simulink model "WaveStar"  (R2018b)
settings: Solver=ode4  StartTime=0  StopTime=141.2  FixedStep=0.001  MaxStep=0.001  RelTol=1e-3  EnableMultiTasking=on
values from neighbouring files (symbols this model uses):
  cc = 10.0    (= 10)    [controller_init.m]
  kc = 0    [controller_init.m]
  L_AB = 0.412    [controller_init.m]
  L_AC = 0.2    [controller_init.m]
  mc = 0    [controller_init.m]
  McSat = inf    [controller_init.m]
  simu = simulationClass()    [wecSimInputFile.m]
  waves = waveClass('irregular')    [wecSimInputFile.m]
  xPcTs = 0.001    [controller_init.m]
undefined symbols (not defined in the file or in its folder): body, constraint, HPfreq, LPfreq, pto, X, Y, Z
libraries: nesl_utility x72, sm_lib x38, WECSim_Lib x7, simulink x2, vrlib x1
(part 4 of 4)

== matlab function WaveStar/Controller/Rotary/lin2rot conversion/Linear2Angular Conversion/MATLAB Function1 K [m] ==
  data: u input; y output; L_AB parameter; L_AC parameter
function y = fcn(u,L_AB,L_AC)
%#codegen
y = L_AB'*L_AC'*sin(u);

== matlab function WaveStar/Controller/Linear/WECCCOMP Controller/lin2rot conversion/Linear2Angular Conversion/MATLAB Function1 a_CAB [rad] ==
  data: u input; y output; L_AB parameter; L_AC parameter
function y = fcn(u,L_AB,L_AC)
%#codegen
%
y = acos((u.^2-L_AB'^2-L_AC'^2)/(-2*L_AB'*L_AC'));

== matlab function WaveStar/C_Revolute/MATLAB Function ==
  data: vel input; t output; brkwy_trq parameter double; brkwy_vel parameter double; Col_trq parameter double; visc_coef parameter double
function t = friction(vel,brkwy_trq, brkwy_vel, Col_trq, visc_coef)
    w = -vel(5);

    %{
    brkwy_trq = .25;         % Breakaway friction torque
    brkwy_vel = 0.1;        % Breakaway friction velocity
    Col_trq = .20;           % Coulomb friction torque
    visc_coef = 0.001;      % Viscous friction coefficient
    %}
    
    static_scale = sqrt(2*exp(1))*(brkwy_trq-Col_trq);  % Scale factor for static torque
    static_thr = sqrt(2)*brkwy_vel;                     % Velocity threshold for static torque
    Col_thr = brkwy_vel/10;                             % Velocity threshold for Coulomb torque
    
    t = visc_coef * w ...
         + static_scale * (w/static_thr*exp(-(w/static_thr)^2)) ...
         + Col_trq * tanh(w/Col_thr);
end

%{
parameters
    brkwy_trq = { 25, 'N*m' };          % Breakaway friction torque
    brkwy_vel = { 0.1, 'rad/s' };       % Breakaway friction velocity
    Col_trq = { 20, 'N*m' };            % Coulomb friction torque
    visc_coef = { 0.001, 'N*m*s/rad' }; % Viscous friction coefficient
end

parameters (Access=private)
    static_scale = sqrt(2*exp(1))*(brkwy_trq-Col_trq);  % Scale factor for static torque
    static_thr = sqrt(2)*brkwy_vel;                     % Velocity threshold for static torque
    Col_thr = brkwy_vel/10;                             % Velocity threshold for Coulomb torque
end

equations
    % Parameter range checking
    assert(brkwy_trq>0)
    assert(brkwy_vel>0)
    assert(Col_trq>0)
    assert(Col_trq<=brkwy_trq)
    assert(visc_coef>=0)
    % Torque is a combination of viscous, static, and Coulomb losses
    t == visc_coef * w ...
         + static_scale * (w/static_thr*exp(-(w/static_thr)^2)) ...
         + Col_trq * tanh(w/Col_thr);
end
%}

== matlab function WaveStar/B_Revolute/MATLAB Function ==
  data: vel input; t output; brkwy_trq parameter double; brkwy_vel parameter double; Col_trq parameter double; visc_coef parameter double
function t = friction(vel,brkwy_trq, brkwy_vel, Col_trq, visc_coef)
    w = -vel(5);

    %{
    brkwy_trq = .25;         % Breakaway friction torque
    brkwy_vel = 0.1;        % Breakaway friction velocity
    Col_trq = .20;           % Coulomb friction torque
    visc_coef = 0.001;      % Viscous friction coefficient
    %}
    
    static_scale = sqrt(2*exp(1))*(brkwy_trq-Col_trq);  % Scale factor for static torque
    static_thr = sqrt(2)*brkwy_vel;                     % Velocity threshold for static torque
    Col_thr = brkwy_vel/10;                             % Velocity threshold for Coulomb torque
    
    t = visc_coef * w ...
         + static_scale * (w/static_thr*exp(-(w/static_thr)^2)) ...
         + Col_trq * tanh(w/Col_thr);
end

%{
parameters
    brkwy_trq = { 25, 'N*m' };          % Breakaway friction torque
    brkwy_vel = { 0.1, 'rad/s' };       % Breakaway friction velocity
    Col_trq = { 20, 'N*m' };            % Coulomb friction torque
    visc_coef = { 0.001, 'N*m*s/rad' }; % Viscous friction coefficient
end

parameters (Access=private)
    static_scale = sqrt(2*exp(1))*(brkwy_trq-Col_trq);  % Scale factor for static torque
    static_thr = sqrt(2)*brkwy_vel;                     % Velocity threshold for static torque
    Col_thr = brkwy_vel/10;                             % Velocity threshold for Coulomb torque
end

equations
    % Parameter range checking
    assert(brkwy_trq>0)
    assert(brkwy_vel>0)
    assert(Col_trq>0)
    assert(Col_trq<=brkwy_trq)
    assert(visc_coef>=0)
    % Torque is a combination of viscous, static, and Coulomb losses
    t == visc_coef * w ...
         + static_scale * (w/static_thr*exp(-(w/static_thr)^2)) ...
         + Col_trq * tanh(w/Col_thr);
end
%}

== matlab function WaveStar/Controller/Rotary/MATLAB Function ==
  data: ws1 input; WS1 output; ws2 input; ws3 input; float_accel input; WS2 output; WS3 output; ACC output; time input; pos input; POS output
function [WS1,WS2,WS3,ACC,POS] = addfault(ws1, ws2, ws3, float_accel, time, pos)
 
%% Wave Gauge 1
bias = 0;
drift = 0;
pDrop = 0.2; %0.3;
x = rand;
rn = 0.002*randn; %0.002*randn;
if x<pDrop
    WS1 = 0;
else
    WS1 = ws1+bias+drift*time+rn;
end
 
%% Wave Gauge 2
bias = 0;
drift = 0;
pDrop = 0.18; %0.15;
x = rand;
rn = 0.002*randn; %0.002*randn;
if x<pDrop
    WS2 = 0;
else
    WS2 = ws2+bias+drift*time+rn;
end

 
%% Wave Gauge 3
bias = 0;
drift = 0;
pDrop = 0.15; %0.2;
x = rand;
rn = 0.002*randn; %0.002*randn;
if x<pDrop
    WS3 = 0;
else
    WS3 = ws3+bias+drift*time+rn;
end
 
%% Accelerometer
bias = 0;
drift = 0;
pDrop = 0.08; %0.23;
x = rand;
rn = 0.25*randn; %0.25*randn;
if x<pDrop
    ACC = 0;
else
    ACC = float_accel+bias+drift*time+rn;
end

%% Position
bias = 0;
drift = 0;
pDrop = 0.03; %0.01;
x = rand;
rn = 0.003*randn; %0.003*randn;

if x<pDrop
    POS = 0;
else
    POS = pos+bias+drift*time+rn;
end

== matlab function WaveStar/A_Revolute/MATLAB Function ==
  data: time input; vel input; t output; brkwy_trq parameter double; brkwy_vel parameter double; Col_trq parameter double; visc_coef parameter double
function t = friction(time,vel,brkwy_trq, brkwy_vel, Col_trq, visc_coef)
    w = -vel(5);

    %{
    brkwy_trq = .25;         % Breakaway friction torque
    brkwy_vel = 0.1;        % Breakaway friction velocity
    Col_trq = .20;           % Coulomb friction torque
    visc_coef = 0.001;      % Viscous friction coefficient
    %}
    
    static_scale = sqrt(2*exp(1))*(brkwy_trq-Col_trq);  % Scale factor for static torque
    static_thr = sqrt(2)*brkwy_vel;                     % Velocity threshold for static torque
    Col_thr = brkwy_vel/10;                             % Velocity threshold for Coulomb torque
    
    if (55 < time)&&(time < 115)
    t = visc_coef * w ...
         + static_scale * (w/static_thr*exp(-(w/static_thr)^2)) ...
         + Col_trq * tanh(w/Col_thr);
    else
        t = 0;
    end
end

%{
parameters
    brkwy_trq = { 25, 'N*m' };          % Breakaway friction torque
    brkwy_vel = { 0.1, 'rad/s' };       % Breakaway friction velocity
    Col_trq = { 20, 'N*m' };            % Coulomb friction torque
    visc_coef = { 0.001, 'N*m*s/rad' }; % Viscous friction coefficient
end

parameters (Access=private)
    static_scale = sqrt(2*exp(1))*(brkwy_trq-Col_trq);  % Scale factor for static torque
    static_thr = sqrt(2)*brkwy_vel;                     % Velocity threshold for static torque
    Col_thr = brkwy_vel/10;                             % Velocity threshold for Coulomb torque
end

equations
    % Parameter range checking
    assert(brkwy_trq>0)
    assert(brkwy_vel>0)
    assert(Col_trq>0)
    assert(Col_trq<=brkwy_trq)
    assert(visc_coef>=0)
    % Torque is a combination of viscous, static, and Coulomb losses
    t == visc_coef * w ...
         + static_scale * (w/static_thr*exp(-(w/static_thr)^2)) ...
         + Col_trq * tanh(w/Col_thr);
end
%}

== matlab function WaveStar/Float/Hydrodynamic Body/Hydrostatic Restoring Force Calculation/Linear and Nonlinear Restoring Force Variant Subsystem/Nonlinear Hydrostatic Restoring Force/Restoring Forces ==
  data: x input; elv input; center input; f output; tnorm input; area input; rho input; g input; cg input; p output; mass input
function [f,p]  = nonLinearBuoyancy(x,elv,center,tnorm,area,rho,g,cg,mass)
% Function to calculate buoyancy force and moment on a triangulated surface
% NOTE: This function assumes that the STL file is imported with its CG at 0,0,0
[f,p] = calc_buoyancy(x,elv,center,tnorm,area,rho,g,cg);
f = -f + [0 0 g*mass 0 0 0]';
end


function [f,p] = calc_buoyancy(x,elv,center,tnorm,area,rho,g,cg)
% Function to apply translation and rotation and calculate forces

% Compute new tri coords after cog rotation and translation
center = rotateXYZ(center,[1 0 0],x(4));
center = rotateXYZ(center,[0 1 0],x(5));
center = rotateXYZ(center,[0 0 1],x(6));
center = offsetXYZ(center,x);
center = offsetXYZ(center,cg);
% Compute new normal vectors coords after cog rotation
tnorm = rotateXYZ(tnorm,[1 0 0],x(4));
tnorm = rotateXYZ(tnorm,[0 1 0],x(5));
tnorm = rotateXYZ(tnorm,[0 0 1],x(6));

% Calculate the hydrostatic forces
av = tnorm .* [area area area];
[f,p]=fHydrostatic(center,elv,x(1:3)+cg,av,rho,g);
end

function verts = offsetXYZ(verts,x)
% Function to move the position vertices
verts(:,1) = verts(:,1) + x(1);
verts(:,2) = verts(:,2) + x(2);
verts(:,3) = verts(:,3) + x(3);
end

function xn = rotateXYZ(x,ax,t)
% Function to rotate a point about an arbitrary axis
% x: 3-componenet coordiantes
% ax: axis about which to rotate (must be a vector length 1)
% t: rotation angle
% xn: new coordinates after rotation
rotMat = zeros(3);
rotMat(1,1) = ax(1)*ax(1)*(1-cos(t))    + cos(t);
rotMat(1,2) = ax(2)*ax(1)*(1-cos(t))    + ax(3)*sin(t);
rotMat(1,3) = ax(3)*ax(1)*(1-cos(t))    - ax(2)*sin(t);
rotMat(2,1) = ax(1)*ax(2)*(1-cos(t))    - ax(3)*sin(t);
rotMat(2,2) = ax(2)*ax(2)*(1-cos(t))    + cos(t);
rotMat(2,3) = ax(3)*ax(2)*(1-cos(t))    + ax(1)*sin(t);
rotMat(3,1) = ax(1)*ax(3)*(1-cos(t))    + ax(2)*sin(t);
rotMat(3,2) = ax(2)*ax(3)*(1-cos(t))    - ax(1)*sin(t);
rotMat(3,3) = ax(3)*ax(3)*(1-cos(t))    + cos(t);
xn = x*rotMat;
end

function [f,p] = fHydrostatic(center,elv,instcg,av,rho,g)
% Function to calculate the force and moment about the cog due to hydrostatic pressure
f = zeros(6,1);

% Zeor out regions above the mean free surface
z=center(:,3); z((z-elv)>0)=0;

% Calculate the hydrostatic pressure at each triangle center
pressureVect = rho*g.*[-z -z -z].*-av;
p = rho*g.*-z;
% Compute force about cog
f(1:3) = sum(pressureVect);

tmp1 = ones(length(center(:,1)),1);
tmp2 = tmp1*instcg';
center2cgVec = center-tmp2;

f(4:6)= sum(cross(center2cgVec,pressureVect));
end

== matlab function WaveStar/Controller/Rotary/lin2rot conversion/Linear2Angular Conversion/MATLAB Function1 L_BC [m] ==
  data: u input; y output; L_BC_neutral parameter
 function y = fcn(u,L_BC_neutral)
%#codegen
%
y = u+L_BC_neutral';

== matlab function WaveStar/Controller/Rotary/lin2rot conversion/Linear2Angular Conversion/MATLAB Function1 Theta [rad] ==
  data: u input; y output; a_CAB_neutral parameter
function y = fcn(u,a_CAB_neutral)
%#codegen
y = u-a_CAB_neutral';

== matlab function WaveStar/Controller/Rotary/lin2rot conversion/Linear2Angular Conversion/MATLAB Function1 a_CAB [rad] ==
  data: u input; y output; L_AB parameter; L_AC parameter
function y = fcn(u,L_AB,L_AC)
%#codegen
%
y = acos((u.^2-L_AB'^2-L_AC'^2)/(-2*L_AB'*L_AC'));

== matlab function WaveStar/Float/Hydrodynamic Body/Morison Element and ViscousDampingForceCalculation/Morison Element Variant Subsystem/Morison Element On/Irregular Wave Morison Force/MorrisonElement(s)  ==
  data: r input; f output; Vel input; Accel input; Disp input; Area input; Cd input; Vol input; Ca input; Time input; rho input; waveDir input; waterDepth input; k input; w input; A input; rampTime input; g input; randPhase input; dw input; currentSpeed input; currentDirection input; currentDepth input; currentOption input
function f = fcn(r,Vel,Accel,Disp,Area,Cd,Vol,Ca,Time,rho,waveDir,waterDepth,k,w,A,rampTime,g,randPhase,dw,currentSpeed,currentDirection,currentDepth,currentOption)
[rr,~]  = size(r); [ff]    = length(w);
FMt     = zeros(rr,6);
uVt     = zeros(ff,1); vVt = uVt; wVt = vVt; uAt = wVt; vAt = uAt; wAt = vAt;
for ii = 1:rr
    % Calculate Rotation Matrix
    RotMax = [cos(Disp(5))*cos(Disp(6)) , cos(Disp(4))*sin(Disp(6)) + sin(Disp(4))*sin(Disp(5))*cos(Disp(6)) , sin(Disp(4))*sin(Disp(6)) - cos(Disp(4))*sin(Disp(5))*sin(Disp(6));...
              -cos(Disp(5))*sin(Disp(6)), cos(Disp(4))*cos(Disp(6)) -  sin(Disp(4))*sin(Disp(5))*sin(Disp(6)), sin(Disp(4))*cos(Disp(6)) + cos(Disp(4))*sin(Disp(5))*sin(Disp(6));...
              sin(Disp(5))              , -sin(Disp(4))*cos(Disp(5))                                         , cos(Disp(4))*cos(Disp(5))                                        ];
    % Rotate Cartesian
    rRot    = mtimes(r(ii,:),RotMax);
    Dispt   = [Disp(1),Disp(2),Disp(3)];
    ShiftCg = Dispt + rRot;
    % Update translational and rotational velocity
    % w refers to \omega = rotational velocity
    Velt    = [Vel(4),Vel(5),Vel(6)];
    wxr     = cross(Velt,r(ii,:));
    %
    switch currentOption
        case 0
            currentSpeedDepth = currentSpeed;
        case 1
            if ShiftCg(3) > -currentDepth
                currentSpeedDepth = currentSpeed*(1 + ShiftCg(3)/currentDepth)^(1/7);
            else
                currentSpeedDepth = 0;
            end
        case 2
            if ShiftCg(3) > -currentDepth
                currentSpeedDepth = currentSpeed*(1 + ShiftCg(3)/currentDepth);
            else
                currentSpeedDepth = 0;
            end
        otherwise
            currentSpeedDepth = 0;
    end
    % Ramp Time
    if Time <= rampTime
        curramp        = currentSpeedDepth*(1 + cos(pi + pi/rampTime*Time))/2;
    else
        curramp        = currentSpeedDepth;
    end
    %Vel should be a column vector
    Vel2    = [Vel(1),Vel(2),Vel(3)] + wxr + [curramp*cosd(currentDirection),curramp*sind(currentDirection),0];
    % Update translational and rotational acceleration
    % dotw refers to \dot{\omega} = rotational acceleration
    Accelt  = [Accel(4),Accel(5),Accel(6)];
    dotwxr  = cross(Accelt,r(ii,:));
    wxwxr   = cross(Velt,wxr);
    % Update Translational Acceleration
    Accel2  = [Accel(1),Accel(2),Accel(3)] + dotwxr + wxwxr;
    %% Calculate Orbital Velocity
    for jj = 1:ff
        waveDirRad      = waveDir*pi/180;
        phaseArg        = w(jj,1)*Time - k(jj,1)*(ShiftCg(1)*cos(waveDirRad) + ShiftCg(2)*sin(waveDirRad)) + randPhase(jj,1);
        % Vertical Variation
        kh              = k(jj,1)*waterDepth;
        kz              = k(jj,1)*ShiftCg(3);
        if kh > pi % Deep Water Wave
            coeffHorz  = exp(kz);
            coeffVert  = coeffHorz;
        else % Shallow & Intermediate depth
            coeffHorz  = cosh(kz + kh)/cosh(kh);
            coeffVert  = sinh(kz + kh)/cosh(kh);
        end
        % Ramp Time
        if Time <= rampTime
            ramp        = (sqrt(A(jj,1)*dw(jj,1))/2)*(1 + cos(pi + pi/rampTime*Time));
        else
            ramp        = sqrt(A(jj,1)*dw(jj,1));
        end
        % Orbital Velocity for each individual wave component
        uVt(jj,1)       =  ramp*coeffHorz*cos(phaseArg)*g*k(jj,1)*(1/w(jj,1))*cos(waveDirRad);
        vVt(jj,1)       =  ramp*coeffHorz*cos(phaseArg)*g*k(jj,1)*(1/w(jj,1))*sin(waveDirRad);
        wVt(jj,1)       = -ramp*coeffVert*sin(phaseArg)*g*k(jj,1)*(1/w(jj,1));
        % Orbital Acceleration for each individual wave component
        uAt(jj,1)       = -ramp*coeffHorz*sin(phaseArg)*g*k(jj,1)*cos(waveDirRad);
        vAt(jj,1)       = -ramp*coeffHorz*sin(phaseArg)*g*k(jj,1)*sin(waveDirRad);
        wAt(jj,1)       = -ramp*coeffVert*cos(phaseArg)*g*k(jj,1);
    end
    % Sum the wave components to obtain the x, y, z orbital velocities
    uV = sum(uVt); uA = sum(uAt); vV = sum(vVt); vA = sum(vAt); wV = sum(wVt); wA = sum(wAt);
    %% Added inertia and drag forces
    areaRot         = abs(mtimes(Area(ii,:),RotMax));
    CdRot           = mtimes(abs(Cd(ii,:)),RotMax);
    CaRot           = abs(mtimes(Ca(ii,:),RotMax));
    % Forces from velocity drag
    uVdiff          = uV - Vel2(1); FxuV = (1/2)*abs(uVdiff)*uVdiff*rho*CdRot(1)*areaRot(1);
    vVdiff          = vV - Vel2(2); FxvV = (1/2)*abs(vVdiff)*vVdiff*rho*CdRot(2)*areaRot(2);
    wVdiff          = wV - Vel2(3); FxwV = (1/2)*abs(wVdiff)*wVdiff*rho*CdRot(3)*areaRot(3);
    % Forces from body acceleration inertia
    uAdiff          = uA - Accel2(1); FxuA = uAdiff*rho*Vol(ii,:)*CaRot(1);
    vAdiff          = vA - Accel2(2); FxvA = vAdiff*rho*Vol(ii,:)*CaRot(2);
    wAdiff          = wA - Accel2(3); FxwA = wAdiff*rho*Vol(ii,:)*CaRot(3);
    % Forces from fluid acceleration inertia
    FxuAf           = uA*Vol(ii,:)*rho;
    FxvAf           = vA*Vol(ii,:)*rho;
    FxwAf           = wA*Vol(ii,:)*rho;
    % Combine the forces and moments
    if ShiftCg(3) > 0
        F           = [0, 0, 0];
        M           = [0, 0, 0];
        FMt(ii,:)   = [F,M];
    else
        F           = [FxuV + FxuA + FxuAf,...
            FxvV + FxvA + FxvAf,...
            FxwV + FxwA + FxwAf];
        M           = cross(rRot,F);
        FMt(ii,:)   = [F,M];
    end
end
f      = 0.* Vel;
f(1:6) = [sum(FMt(:,1));sum(FMt(:,2));sum(FMt(:,3));sum(FMt(:,4));sum(FMt(:,5));sum(FMt(:,6))];

== matlab function WaveStar/Float/Hydrodynamic Body/Morison Element and ViscousDampingForceCalculation/Morison Element Variant Subsystem/Morison Element On/No Wave Morison Force/MorrisonElement(s)  ==
  data: r input; f output; Vel input; Accel input; Disp input; Area input; Cd input; Vol input; Ca input; rho input; currentSpeed input; currentDirection input; Time input; rampTime input; currentDepth input; currentOption input
function f = fcn(r,Vel,Accel,Disp,Area,Cd,Vol,Ca,rho,currentSpeed,currentDirection,Time,rampTime,currentDepth,currentOption)
[rr,~]=size(r);
FMt = zeros(rr,6);
for ii = 1:rr
    % Calculate Rotation Matrix
    RotMax = [cos(Disp(5))*cos(Disp(6)) , cos(Disp(4))*sin(Disp(6)) + sin(Disp(4))*sin(Disp(5))*cos(Disp(6)) , sin(Disp(4))*sin(Disp(6)) - cos(Disp(4))*sin(Disp(5))*sin(Disp(6));...
             -cos(Disp(5))*sin(Disp(6)), cos(Disp(4))*cos(Disp(6)) -  sin(Disp(4))*sin(Disp(5))*sin(Disp(6)), sin(Disp(4))*cos(Disp(6)) + cos(Disp(4))*sin(Disp(5))*sin(Disp(6));...
              sin(Disp(5))              , -sin(Disp(4))*cos(Disp(5))                                         , cos(Disp(4))*cos(Disp(5))                                        ];
    % Rotate Cartesian
    rRot    = mtimes(r(ii,:),RotMax);
    Dispt   = [Disp(1),Disp(2),Disp(3)];
    ShiftCg = Dispt + rRot;
    % Update translational and rotational velocity
    Velt    = [Vel(4),Vel(5),Vel(6)];                       % w refers to \omega = rotational velocity
    wxr     = cross(Velt,r(ii,:));
    switch currentOption
        case 0
             currentSpeedDepth = currentSpeed;
        case 1
            if ShiftCg(3) > -currentDepth
                currentSpeedDepth = currentSpeed*(1 + ShiftCg(3)/currentDepth)^(1/7);
            else
                currentSpeedDepth = 0;
            end
        case 2
            if ShiftCg(3) > -currentDepth
                currentSpeedDepth = currentSpeed*(1 + ShiftCg(3)/currentDepth);
            else
                currentSpeedDepth = 0;
            end
        otherwise
             currentSpeedDepth = 0;
    end
    % Ramp Time
    if Time <= rampTime
            curramp        = currentSpeedDepth*(1 + cos(pi + pi/rampTime*Time))/2;
        else
            curramp        = currentSpeedDepth;
    end
    %Vel should be a column vector
    Vel2    = [Vel(1),Vel(2),Vel(3)] + wxr + [curramp*cosd(currentDirection),curramp*sind(currentDirection),0];
    % Update translational and rotational acceleration
    Accelt  = [Accel(4),Accel(5),Accel(6)];
    dotwxr  = cross(Accelt,r(ii,:));                        % dotw refers to \dot{\omega} = rotational acceleration
    wxwxr   = cross(Velt,wxr);
    Accel2  = [Accel(1),Accel(2),Accel(3)] + dotwxr + wxwxr;
    %% Added inertia and drag forces
    areaRot = abs(mtimes(Area(ii,:),RotMax));
    CdRot   = mtimes(abs(Cd(ii,:)),RotMax);
    CaRot   = abs(mtimes(Ca(ii,:),RotMax));
    % Forces from body velocity drag
    FxuV    = (1/2)*abs(-1*Vel2(1))*-1*Vel2(1)*rho*CdRot(1)*areaRot(1);
    FxvV    = (1/2)*abs(-1*Vel2(2))*-1*Vel2(2)*rho*CdRot(2)*areaRot(2);
    FxwV    = (1/2)*abs(-1*Vel2(3))*-1*Vel2(3)*rho*CdRot(3)*areaRot(3);
    % Forces from body acceleration inertia
    FxuA = rho*Vol(ii,:)*CaRot(1)*-1*Accel2(1);
    FxvA = rho*Vol(ii,:)*CaRot(2)*-1*Accel2(2);
    FxwA = rho*Vol(ii,:)*CaRot(3)*-1*Accel2(3);
    % Sum the force and moment contributions
    if ShiftCg(3) > 0
        FMt(ii,:)   = [0, 0, 0, 0, 0, 0];
    else
        F           = [FxuV + FxuA,...
            FxvV + FxvA,...
            FxwV + FxwA];
        M           = cross(rRot,F);
        FMt(ii,:)   = [F,M];
    end
end
f      = 0.*Vel;
f(1:6) = [sum(FMt(:,1));sum(FMt(:,2));sum(FMt(:,3));sum(FMt(:,4));sum(FMt(:,5));sum(FMt(:,6))];

== matlab function WaveStar/Float/Hydrodynamic Body/Morison Element and ViscousDampingForceCalculation/Morison Element Variant Subsystem/Morison Element On/Regular Wave Morison Force/MorrisonElement(s)  ==
  data: r input; f output; Vel input; Accel input; Disp input; Area input; Cd input; Vol input; Ca input; Time input; rho input; waveDir input; waterDepth input; k input; w input; A input; rampTime input; g input; currentSpeed input; currentDirection input; currentDepth input; currentOption input
function f = fcn(r,Vel,Accel,Disp,Area,Cd,Vol,Ca,Time,rho,waveDir,waterDepth,k,w,A,rampTime,g,currentSpeed,currentDirection,currentDepth,currentOption)
[rr,~]=size(r);
FMt = zeros(rr,6);
for ii = 1:rr
    % Calculate Rotation Matrix
    RotMax = [cos(Disp(5))*cos(Disp(6)) , cos(Disp(4))*sin(Disp(6)) + sin(Disp(4))*sin(Disp(5))*cos(Disp(6)) , sin(Disp(4))*sin(Disp(6)) - cos(Disp(4))*sin(Disp(5))*sin(Disp(6));...
             -cos(Disp(5))*sin(Disp(6)), cos(Disp(4))*cos(Disp(6)) -  sin(Disp(4))*sin(Disp(5))*sin(Disp(6)), sin(Disp(4))*cos(Disp(6)) + cos(Disp(4))*sin(Disp(5))*sin(Disp(6));...
              sin(Disp(5))              , -sin(Disp(4))*cos(Disp(5))                                         , cos(Disp(4))*cos(Disp(5))                                        ];
    % Rotate Cartesian
    rRot    = mtimes(r(ii,:),RotMax);
    Dispt   = [Disp(1),Disp(2),Disp(3)];
    ShiftCg = Dispt + rRot;
    % Update translational and rotational velocity
    % w refers to \omega = rotational velocity
    Velt    = [Vel(4),Vel(5),Vel(6)]; 
    wxr     = cross(Velt,r(ii,:));
    %
    switch currentOption
        case 0
             currentSpeedDepth = currentSpeed;
        case 1
            if ShiftCg(3) > -currentDepth
                currentSpeedDepth = currentSpeed*(1 + ShiftCg(3)/currentDepth)^(1/7);
            else
                currentSpeedDepth = 0;
            end
        case 2
            if ShiftCg(3) > -currentDepth
                currentSpeedDepth = currentSpeed*(1 + ShiftCg(3)/currentDepth);
            else
                currentSpeedDepth = 0;
            end
        otherwise
             currentSpeedDepth = 0;
    end
    % Ramp Time
    if Time <= rampTime
            curramp        = currentSpeedDepth*(1 + cos(pi + pi/rampTime*Time))/2;
        else
            curramp        = currentSpeedDepth;
    end
    %Vel should be a column vector
    Vel2    = [Vel(1),Vel(2),Vel(3)] + wxr + [curramp*cosd(currentDirection),curramp*sind(currentDirection),0];
    % Update translational and rotational acceleration
    % dotw refers to \dot{\omega} = rotational acceleration
    Accelt  = [Accel(4),Accel(5),Accel(6)];
    dotwxr  = cross(Accelt,r(ii,:));
    wxwxr   = cross(Velt,wxr);
    Accel2  = [Accel(1),Accel(2),Accel(3)] + dotwxr + wxwxr;
    %% Calculate Orbital Velocity
    waveDirRad     = waveDir*pi/180;
    phaseArg       = w*Time - k*(ShiftCg(1)*cos(waveDirRad) + ShiftCg(2)*sin(waveDirRad));
    % Vertical Variation
    kh              = k*waterDepth;
    kz              = k*ShiftCg(3);
    if kh > pi  % Deep water wave
        coeffHorz  = exp(kz);
        coeffVert  = coeffHorz;
    else        % Shallow & Intermediate Depth
        coeffHorz  = cosh(kz + kh)/cosh(kh);
        coeffVert  = sinh(kz + kh)/cosh(kh);
    end
    % Ramp Time
    if Time <= rampTime
        ramp        = (A/2)*(1 + cos( pi + pi/rampTime*Time));
    else
        ramp        = A;
    end
    % Orbital Velocity
    uV              =  ramp*coeffHorz*cos(phaseArg)*g*k*(1/w)*cos(waveDirRad);
    vV              =  ramp*coeffHorz*cos(phaseArg)*g*k*(1/w)*sin(waveDirRad);
    wV              = -ramp*coeffVert*sin(phaseArg)*g*k*(1/w);
    % Orbital Acceleration
    uA              = -ramp*coeffHorz*sin(phaseArg)*g*k*cos(waveDirRad);
    vA              = -ramp*coeffHorz*sin(phaseArg)*g*k*sin(waveDirRad);
    wA              = -ramp*coeffVert*cos(phaseArg)*g*k;
    %% Added inertia and drag forces
    areaRot         = abs(mtimes(Area(ii,:),RotMax));
    CdRot           = mtimes(abs(Cd(ii,:)),RotMax);
    CaRot           = abs(mtimes(Ca(ii,:),RotMax));
    % Forces from velocity drag
    uVdiff          = uV - Vel2(1); FxuV = (1/2)*abs(uVdiff)*uVdiff*rho*CdRot(1)*areaRot(1);
    vVdiff          = vV - Vel2(2); FxvV = (1/2)*abs(vVdiff)*vVdiff*rho*CdRot(2)*areaRot(2);
    wVdiff          = wV - Vel2(3); FxwV = (1/2)*abs(wVdiff)*wVdiff*rho*CdRot(3)*areaRot(3);
    % Forces from body acceleration inertia
    uAdiff          = uA - Accel2(1); FxuA = uAdiff*rho*Vol(ii,:)*CaRot(1);
    vAdiff          = vA - Accel2(2); FxvA = vAdiff*rho*Vol(ii,:)*CaRot(2);
    wAdiff          = wA - Accel2(3); FxwA = wAdiff*rho*Vol(ii,:)*CaRot(3);
    % Forces from fluid acceleration inertia
    FxuAf           = uA*Vol(ii,:)*rho;
    FxvAf           = vA*Vol(ii,:)*rho;
    FxwAf           = wA*Vol(ii,:)*rho;
    % Sum the three force contributions
    if ShiftCg(3) > 0
        F           = [0, 0, 0];
        M           = [0, 0, 0];
        FMt(ii,:)   = [F,M];
    else
        F           = [FxuV + FxuA + FxuAf,...
            FxvV + FxvA + FxvAf,...
            FxwV + FxwA + FxwAf];
        M           = cross(rRot,F);
        FMt(ii,:)   = [F,M];
    end
end
f      = 0.*Vel;
f(1:6) = [sum(FMt(:,1));sum(FMt(:,2));sum(FMt(:,3));sum(FMt(:,4));sum(FMt(:,5));sum(FMt(:,6))];

== matlab function WaveStar/Float/Hydrodynamic Body/Nonlinear Wave Elevation/Linear or Instantaneous Free Surface/Instantaneous Water Free Surface  /Instantaneous FS ==
  data: x input; center input; f output; cg input; AH input; w input; dw input; k input; typeNum input; t input; rampT input; phaseRand input; waveDir input
function f  = waveElevation(x,center,cg,AH,w,dw,k,typeNum,t,rampT,phaseRand,waveDir)
% Function to calculate the wave elevation at the ceontroids of triangulated surface
% NOTE: This function assumes that the STL file is imported with its CG at 0,0,0
f = calc_elev(x,center,cg,AH,w,dw,k,typeNum,t,rampT,phaseRand, waveDir);
end

function f = calc_elev(x,center,cg,AH,w,dw,k,typeNum,t,rampT,phaseRand,waveDir)
% Function to rotate and translate body and call wave elevation function at new locations

% Compute new tri center coords after cog rotation and translation
center = rotateXYZ(center,[1 0 0],x(4));
center = rotateXYZ(center,[0 1 0],x(5));
center = rotateXYZ(center,[0 0 1],x(6));
center = offsetXYZ(center,x);
center = offsetXYZ(center,cg);
% Calculate the free surface
f=waveElev(center,AH,w,dw,t,k,rampT,phaseRand,typeNum,waveDir);
end

function verts = offsetXYZ(verts,x)
% Function to move the position vertices
verts(:,1) = verts(:,1) + x(1);
verts(:,2) = verts(:,2) + x(2);
verts(:,3) = verts(:,3) + x(3);
end

function xn = rotateXYZ(x,ax,t)
% Function to rotate a point about an arbitrary axis
% x: 3-component coordinates
% ax: axis about which to rotate (must be a vector length 1)
% t: rotation angle
% xn: new coordinates after rotation
rotMat = zeros(3);
rotMat(1,1) = ax(1)*ax(1)*(1-cos(t))    + cos(t);
rotMat(1,2) = ax(2)*ax(1)*(1-cos(t))    + ax(3)*sin(t);
rotMat(1,3) = ax(3)*ax(1)*(1-cos(t))    - ax(2)*sin(t);
rotMat(2,1) = ax(1)*ax(2)*(1-cos(t))    - ax(3)*sin(t);
rotMat(2,2) = ax(2)*ax(2)*(1-cos(t))    + cos(t);
rotMat(2,3) = ax(3)*ax(2)*(1-cos(t))    + ax(1)*sin(t);
rotMat(3,1) = ax(1)*ax(3)*(1-cos(t))    + ax(2)*sin(t);
rotMat(3,2) = ax(2)*ax(3)*(1-cos(t))    - ax(1)*sin(t);
rotMat(3,3) = ax(3)*ax(3)*(1-cos(t))    + cos(t);
xn = x*rotMat;
end

function f=waveElev(center,AH,w,dw,t,k,rampT,phaseRand,typeNum,waveDir)
% Function to calculate the wave elevation at an array of points
f = zeros(length(center(:,3)),1);
cx = center(:,1);
cy = center(:,2);
X = cx*cos(waveDir*pi/180) + cy*sin(waveDir*pi/180);
if typeNum <10
elseif typeNum <20
    f = AH(1).*cos(k(1).*X-w(1)*t);
elseif typeNum <30
    tmp=sqrt(AH.*dw);
    tmp1 = ones(1,length(center(:,1)));
    tmp2 = (w.*t+phaseRand)*tmp1;
    tmp3 = cos(k*X'- tmp2);
    f(:,1) = tmp3'*tmp;
end
if t<=rampT
    rampF = (1+cos(pi+pi*t/rampT))/2;
    f = f.*rampF;
end
end

== matlab function WaveStar/Float/Hydrodynamic Body/Structure/Motion Sensor/Angle ==
  data: Q input; E output
function E  = EulerAngle(Q)
% Euler Angle Type II or Tait-Bryan Angle for sequence 321 or zyx (Nautical or Cardan angles).
% Yaw [-180,180], followed by pitch [-90,90], followed by roll [-180,180]
E = zeros(3,1);
E(1) = atan2((2*(Q(1)*Q(2)+Q(3)*Q(4))),(1-2*(Q(2)^2+Q(3)^2)));
E(2) = asin(2*(Q(1)*Q(3)-Q(4)*Q(2)));
E(3) = atan2((2*(Q(1)*Q(4)+Q(2)*Q(3))),(1-2*(Q(3)^2+Q(4)^2)));

== matlab function WaveStar/Float/Hydrodynamic Body/Wave Diffraction and Excitation Force Calculation/Linear Wave Excitation Force Variant Subsystem/Irregular Wave Excitation Force/MATLAB Function ==
  data: A input; Fext output; w input; fExtRE input; fExtIM input; phaseRand input; dw input; time input; WaveDir input; WaveSpread input; fExtMD input
function Fext = fcn(A,w,fExtRE,fExtIM,phaseRand,dw,time,WaveDir,WaveSpread,fExtMD)
%#codegen

% pversistent A1 B1 B11 C1 D1 D11 E1 E11

A1=bsxfun(@plus,w*time,pi/2);
Fext = zeros(1,6);
for ii=1:length(WaveDir)
    B1= sin(bsxfun(@plus,A1,phaseRand(:,ii)));
    B11 = sin(bsxfun(@plus,w*time,phaseRand(:,ii)));
    C0 = bsxfun(@times,A*WaveSpread(ii),dw);
    C1 = sqrt(bsxfun(@times,A*WaveSpread(ii),dw));
    D0 =bsxfun(@times,squeeze(fExtMD(ii,:,:)),C0);
    D1 =bsxfun(@times,squeeze(fExtRE(ii,:,:)),C1);
    D11 = bsxfun(@times,squeeze(fExtIM(ii,:,:)),C1);
    E1 = D0+ bsxfun(@times,B1,D1);
    E11 = bsxfun(@times,B11,D11);
    Fext = Fext + sum(bsxfun(@minus,E1,E11));
end

== matlab function WaveStar/Float/Hydrodynamic Body/Wave Diffraction and Excitation Force Calculation/Nonlinear FK Force Variant Subsystem/With Nonlinear FroudeKrylov Force/Diffraction and Excitation Forces ==
  data: x input; elv input; center input; f output; tnorm input; area input; rho input; g input; cg input; AH input; w input; dw input; wDepth input; deepWaterWave input; k input; typeNum input; t input; phaseRand input; wp output; wpMeanFS output
function [f, wp, wpMeanFS]  = nonFKForce(x,elv,center,tnorm,area,rho,g,cg,AH,w,dw,wDepth,deepWaterWave,k,typeNum,t,phaseRand)
% Function to calculate wave exitation force and moment on a triangulated surface
% NOTE: This function assumes that the STL file is imported with its CG at 0,0,0

% Logic to calculate nonFKForce at reduced sample time
[f, wp, wpMeanFS] = calc_force(x,elv,center,tnorm,area,rho,g,cg,AH,w,dw,wDepth,deepWaterWave,k,typeNum,t,phaseRand);
end

function [f, wp, wpMeanFS]  = calc_force(x,elv,center,tnorm,area,rho,g,cg,AH,w,dw,wDepth,deepWaterWave,k,typeNum,t,phaseRand)
% Function to apply translation and rotation, and calculate forces.

% Compute new tri coords after cog rotation and translation
centerMeanFS = offsetXYZ(center,cg);
avMeanFS     = tnorm .* [area area area];

% Compute new tri coords after cog rotation and translation
center = rotateXYZ(center,[1 0 0],x(4));
center = rotateXYZ(center,[0 1 0],x(5));
center = rotateXYZ(center,[0 0 1],x(6));
center = offsetXYZ(center,x);
center = offsetXYZ(center,cg);
% Compute new normal vectors coords after cog rotation and translation
tnorm = rotateXYZ(tnorm,[1 0 0],x(4));
tnorm = rotateXYZ(tnorm,[0 1 0],x(5));
tnorm = rotateXYZ(tnorm,[0 0 1],x(6));

% Copute area vectors
av = tnorm .* [area area area];

% Calculate the free surface
wpMeanFS=pDis(centerMeanFS,       0,AH,w,dw,wDepth,deepWaterWave,t,k,phaseRand,typeNum,rho,g);
wp      =pDis(center      ,     elv,AH,w,dw,wDepth,deepWaterWave,t,k,phaseRand,typeNum,rho,g);

% Calculate forces
f_linear   =FK(centerMeanFS,       cg,avMeanFS,wpMeanFS);
f_nonLinear=FK(center      ,x(1:3)+cg,av      ,wp      );
f = f_nonLinear-f_linear;
end

function verts = offsetXYZ(verts,x)
% Function to move the position vertices
verts(:,1) = verts(:,1) + x(1);
verts(:,2) = verts(:,2) + x(2);
verts(:,3) = verts(:,3) + x(3);
end

function xn = rotateXYZ(x,ax,t)
% Function to rotate a point about an arbitrary axis
% x: 3-componenet coordinates
% ax: axis about which to rotate (must be a vector length 1)
% t: rotation angle
% xn: new coordinates after rotation
rotMat = zeros(3);
rotMat(1,1) = ax(1)*ax(1)*(1-cos(t))    + cos(t);
rotMat(1,2) = ax(2)*ax(1)*(1-cos(t))    + ax(3)*sin(t);
rotMat(1,3) = ax(3)*ax(1)*(1-cos(t))    - ax(2)*sin(t);
rotMat(2,1) = ax(1)*ax(2)*(1-cos(t))    - ax(3)*sin(t);
rotMat(2,2) = ax(2)*ax(2)*(1-cos(t))    + cos(t);
rotMat(2,3) = ax(3)*ax(2)*(1-cos(t))    + ax(1)*sin(t);
rotMat(3,1) = ax(1)*ax(3)*(1-cos(t))    + ax(2)*sin(t);
rotMat(3,2) = ax(2)*ax(3)*(1-cos(t))    - ax(1)*sin(t);
rotMat(3,3) = ax(3)*ax(3)*(1-cos(t))    + cos(t);
xn = x*rotMat;
end

function f=pDis(center,elv,AH,w,dw,wDepth,deepWaterWave,t,k,phaseRand,typeNum,rho,g)
% Function to calculate pressure distribution
f = zeros(length(center(:,3)),1);
z=zeros(length(center(:,1)),1);
if typeNum <10
elseif typeNum <20
    f = rho.*g.*AH(1).*cos(k(1).*center(:,1)-w(1)*t);
    if deepWaterWave == 0
        z=(center(:,3)-elv).*wDepth./(wDepth+elv);
        f = f.*(cosh(k(1).*(z+wDepth))./cosh(k(1)*wDepth));
    else
        z=(center(:,3)-elv);
        f = f.*exp(k(1).*z);
    end
elseif typeNum <30
    for i=1:length(AH)
        if deepWaterWave == 0 && wDepth <= 0.5*pi/k(i)
            z=(center(:,3)-elv).*wDepth./(wDepth+elv);
            f_tmp = rho.*g.*sqrt(AH(i)*dw(i)).*cos(k(i).*center(:,1)-w(i)*t-phaseRand(i));
            f = f + f_tmp.*(cosh(k(i).*(z+wDepth))./cosh(k(i).*wDepth));
        else
            z=(center(:,3)-elv);
            f_tmp = rho.*g.*sqrt(AH(i)*dw(i)).*cos(k(i).*center(:,1)-w(i)*t-phaseRand(i));
            f = f + f_tmp.*exp(k(i).*z);
        end
    end
end
f(z>0)=0;
end

function f = FK(center,instcg,av,wp)
% Function to calculate the force and moment about the cog due to Froude-Krylov pressure
f = zeros(6,1);

% Calculate the hydrostatic pressure at each triangle center
pressureVect = [wp wp wp].*-av;

% Compute force about cog
f(1:3) = sum(pressureVect);

% Compute moment about cog
tmp1 = ones(length(center(:,1)),1);
tmp2 = tmp1*instcg';
center2cgVec = center-tmp2;

f(4:6)= sum(cross(center2cgVec,pressureVect));
end

== matlab function WaveStar/Float/Hydrodynamic Body/Wave Radiation Forces Calculation/SS CI and Constant-Damping-CoeVariant Subsystem/Convolution Integral Calculation/MATLAB Function1 ==
  data: v input; F_FM output; IRKB input; lenJ input; CTTime input
function F_FM = ConvolutionIntegral_interp(v, IRKB, lenJ, CTTime)
%#codegen
% Function to calculate convolution integral

%define persistent variables
interp_factor = 1;
persistent velocity IRKB_interp CTTime_interp;

if isempty(velocity) 
    CTTime_interp  = CTTime(1:interp_factor:end);
    velocity       = zeros(lenJ,length(CTTime_interp));
    IRKB_reordered = permute(IRKB,[3 1 2]);                     % permutes from [601 6 12] to [12 601 6]
    IRKB_interp    = IRKB_reordered(:,1:interp_factor:end, :);  % what does this do?
end 
% shift velocity
velocity      = circshift(velocity, 1, 2);
v = v(:)'';           %force v to be a column
velocity(:,1) = v(:);

%integrate
time_series = bsxfun(@times, IRKB_interp, velocity);
F_FM = squeeze(trapz(CTTime_interp,sum(time_series, 1)));

end

== matlab function WaveStar/Float/Non-Hydro Body/Structure/Motion Sensor/Angle ==
  data: Q input; E output
function E  = EulerAngle(Q)
% Euler Angle Type II or Tait-Bryan Angle for sequence 321 or zyx (Nautical or Cardan angles).
% Yaw [-180,180], followed by pitch [-90,90], followed by roll [-180,180]
E = zeros(3,1);
E(1) = atan2( (2*(Q(1)*Q(2)+Q(3)*Q(4))), (1-2* (Q(2)^2+Q(3)^2) ) );
E(2) = asin( 2* (Q(1)*Q(3) - Q(4)*Q(2)));
E(3) = atan2( (2*(Q(1)*Q(4)+Q(2)*Q(3))), (1-2* (Q(3)^2+Q(4)^2) ) );
